simulink model "arducopter"  (R2021a)
settings: Solver=FixedStepAuto  StartTime=0.0  StopTime=simIn.param.timeEnd  FixedStep=simIn.param.dt  RelTol=1e-3
undefined symbols (not defined in the file or in its folder): DiscIntNeverNeededParam, sim, simIn
libraries: simulink x35, slident x4, vrlib x1
(part 8 of 9)

== matlab function arducopter/Lowpass2p/Lowpass Yaw/Lowpass2p ==
  data: u input; y output; sampleFreq input; cutoffFreq input; delElem1 data_store_memory; delElem2 data_store_memory
function y = lowpass2p(u, sampleFreq, cutoffFreq)
% Lowpass filter of order two
% Source: LowPassFilter2p.cpp
global delElem1
global delElem2

% Calculate parameters: LowPassFilter2p.cpp, compute_params()
fr = single(sampleFreq/cutoffFreq);
ohm = single(tan(pi/fr));
c = single(1+2*cos(pi/4)*ohm + ohm*ohm);

b0 = ohm*ohm/c;
b1 = 2*b0;
b2 = b0;
a1 = 2*(ohm*ohm-1)/c;
a2 = single((1-2*cos(pi/4)*ohm+ohm*ohm)/c);

% Calculation of filtered sample: LowPassFilter2p.cpp, apply()
delElem0 = u - delElem1 * a1 - delElem2 * a2;
y = delElem0 * b0 + delElem1 * b1 + delElem2 * b2;

delElem2 = delElem1;
delElem1 = delElem0;

== matlab function arducopter/Body Frame Rates -> DCM/MATLAB Function ==
  data: dcm input; quaternion output
function quaternion = from_rotation_matrix(dcm)
% Function to calculate quaternion from a given rotation matrix.
% Implemented based on QuaternionT<T>::from_rotation_matrx()

m00 = dcm(1,1);
m11 = dcm(2,2);
m22 = dcm(3,3);
m10 = dcm(2,1);
m01 = dcm(1,2);
m20 = dcm(3,1);
m02 = dcm(1,3);
m21 = dcm(3,2);
m12 = dcm(2,3);

tr = m00 + m11 + m22;

if tr > 0
    S = sqrt(tr+1) * 2;
    qw = 0.25 * S;
    qx = (m21 - m12) / S;
    qy = (m02 - m20) / S;
    qz = (m10 - m01) / S;
elseif ((m00 > m11) && (m00 > m22))
    S = sqrt(1.0 + m00 - m11 - m22) * 2.0;
    qw = (m21 - m12) / S;
    qx = 0.25 * S;
    qy = (m01 + m10) / S;
    qz = (m02 + m20) / S;
elseif (m11 > m22)
    S = sqrt(1.0 + m11 - m00 - m22) * 2.0;
    qw = (m02 - m20) / S;
    qx = (m01 + m10) / S;
    qy = 0.25 * S;
    qz = (m12 + m21) / S;
else
    S = sqrt(1.0 + m22 - m00 - m11) * 2.0;
    qw = (m10 - m01) / S;
    qx = (m02 + m20) / S;
    qy = (m12 + m21) / S;
    qz = 0.25 * S;
end

quaternion = [qw;qx;qy;qz];

== matlab function arducopter/Attitude Controller/MATLAB Function ==
  data: rollIn input; rollOut output; pitchIn input; angleMax input; angleLimit input; pitchOut output; rpyInputMax input
function [rollOut, pitchOut] = get_pilot_desired_lean_angles(rollIn, pitchIn, angleMax, angleLimit, rpyInputMax)
% Code based on Mode::get_pilot_desired_lean_angles()
% Transform pilot's roll and pitch input into desired lean angle in
% centi-degrees

% Calculate inputs to rc_input_to_roll_pitch() function
rollInUnit = rollIn / rpyInputMax;
pitchInUnit = pitchIn / rpyInputMax;
angleMax = angleMax / 100;
angleLimit = angleLimit / 100;

%% The following lines result from the call to rc_input_to_roll_pitch() (control.cpp)
angleMaxDeg = min(angleMax, 85);
rc2rad = angleMaxDeg * pi / 180;

% Convert roll and pitch stick positions to normalized horizontal thrust
thrust_x = -1 * tan(rc2rad * pitchInUnit);
thrust_y = tan(rc2rad * rollInUnit);

% Calculate the horizontal thrust limit based on the angle limit
angleLimit = min( max( 10, angleLimit), angleMaxDeg);
thrustLimit = tan(angleLimit * pi / 180);

% Apply horizontal thrust limit - Lines are taken from
% Vector2<T>::limit_length() and limit thrust vector norm
thrustVecLength = sqrt(thrust_x^2 + thrust_y^2);
if thrustVecLength > thrustLimit && thrustVecLength > 0
   thrust_x = thrust_x * (thrustLimit / thrustVecLength);
   thrust_y = thrust_y * (thrustLimit / thrustVecLength);
end

% Conversion from angular thrust to euler angles
pitchRad = (-1) * atan(thrust_x);
rollRad = atan(cos(pitchRad) * thrust_y);

% Output values in centi-degrees
pitchOut = pitchRad * (100 * 180) / pi;
rollOut = rollRad * (100 * 180) / pi;

== matlab function arducopter/Attitude Controller/MATLAB Function1 ==
  data: yawIn input; yawOut output; pilotYawExpo input; pilotYawRate input
function yawOut = get_pilot_desired_yaw_rate(yawIn, pilotYawExpo, pilotYawRate)
% Code taken from Mode::get_pilot_desired_yaw_rate()
% Transforms pilot's yaw input into a desired yaw rate

%% 1) Apply expo - Code based on input_expo in control.cpp
yawIn = min(max(yawIn, -1), 1);
if pilotYawExpo < 0.95
    yawIn = (1 - pilotYawExpo) * yawIn / (1 - pilotYawExpo * abs(yawIn));
end

%% 2) Convert pilot input to the desired yaw rate
yawOut = pilotYawRate * 100 * yawIn;

== matlab function arducopter/Attitude Controller/input_euler_angle_roll_pitch_euler_rate_yaw()/MATLAB Function ==
  data: q input; roll output; pitch output; yaw output
function [roll, pitch, yaw] = toEuler(q)
% Function takes a quaternion and translates it into Euler angles
% Based on QuaternionT<T>::to_euler() and incorporates 
% QuaternionT<T>::get_euler_roll(), QuaternionT<T>::get_euler_pitch() and
% QuaternionT<T>::get_euler_yaw()

roll = single(atan2(2 * (q(1)*q(2) + q(3)*q(4)), 1 - 2*(q(2)*q(2) + q(3)*q(3))));
% Check if argument of asin is greater than 1 oder smaller than -1
% Based on safe_asin() in AP_MATH.cpp
xPitch = 2 * (q(1)*q(3) - q(4)*q(2));
if xPitch >= 1
    pitch = single(pi/2);
elseif xPitch <= -1
    pitch = single(-pi/2);
else
    pitch = single(asin(xPitch));
end
yaw = single(atan2(2*(q(1)*q(4) + q(2)*q(3)), 1 - 2*(q(3)*q(3) + q(4)*q(4))));

== matlab function arducopter/Attitude Controller/input_euler_angle_roll_pitch_euler_rate_yaw()/Feedforward enabled/MATLAB Function ==
  data: eulerAngleTar input; eulerAccelMaxBF output; eulerAccelMaxEF input
function eulerAccelMaxBF = euler_accel_limit(eulerAngleTar, eulerAccelMaxEF)
% Translation of acceleration limits eulerAccelMax to the euler axis
% Code based on AC_AttitudeControl::euler_accel_limit()

sin_phi = max(min(abs(single(sin(eulerAngleTar(1)))), 1), 0.1); % Sinus of roll angle
cos_phi = max(min(abs(single(cos(eulerAngleTar(1)))), 1), 0.1);
sin_theta = max(min(abs(single(sin(eulerAngleTar(2)))), 1), 0.1); % Sinus of pitch angle

eulerAccelMaxBF = single(zeros(3,1));
if eulerAccelMaxEF(1) == 0 || eulerAccelMaxEF(2) == 0 || eulerAccelMaxEF(3) == 0 || ...
   eulerAccelMaxEF(1) < 0 || eulerAccelMaxEF(2) < 0 || eulerAccelMaxEF(3) < 0 
    eulerAccelMaxBF(1) = eulerAccelMaxEF(1);
    eulerAccelMaxBF(2) = eulerAccelMaxEF(2);
    eulerAccelMaxBF(3) = eulerAccelMaxEF(3);
else
    eulerAccelMaxBF(1) = eulerAccelMaxEF(1);
    eulerAccelMaxBF(2) = min(eulerAccelMaxEF(2) / cos_phi, eulerAccelMaxEF(3) / sin_phi);
    eulerAccelMaxBF(3) = min(min(eulerAccelMaxEF(1) / sin_theta, eulerAccelMaxEF(2) / sin_phi), eulerAccelMaxEF(3) / cos_phi);
end

== matlab function arducopter/Attitude Controller/input_euler_angle_roll_pitch_euler_rate_yaw()/Feedforward enabled/input shaping/input shaping roll angle/Square Root Controller ==
  data: err input; correction_rate output; p input; second_ord_lim input; dt input
function correction_rate = sqrt_controller(err, p, second_ord_lim, dt)
% The square root controller
% Code is taken from sqrt_controller(...) in AC_PosControl.cpp, line 296.

if (second_ord_lim < 0 || second_ord_lim == 0)
   correction_rate = err * p;
elseif (p == 0)
    % P term is zero, but second order limit is positive
    if (err > 0)
        correction_rate = sqrt(single(2.0) * second_ord_lim * err);
    elseif (err < 0)
        correction_rate = sqrt(single(2.0) * second_ord_lim * -err);
    else
        correction_rate = single(0.0);
    end
else
    % P term and second order limit are positive, hence have been defined
    linear_dist = second_ord_lim / (p * p);
    % Check if error exceeds linear range of controller gain
    if (err > linear_dist)
        correction_rate = sqrt(single(2.0) * second_ord_lim * ( err - (linear_dist / single(2.0)) ));
    elseif (err < -linear_dist)
        correction_rate = -sqrt(single(2.0) * second_ord_lim * ( -err - (linear_dist / single(2.0)) ));
    else
        % Return linearly amplified correction if error is in linear range
        correction_rate = err * p;
    end
end

% Prevent oscillations by over-shooting the error correction in the last
% time step
if (dt ~= 0)
    correction_rate = max( min(correction_rate, abs(err) / dt), -abs(err) / dt);
end

== matlab function arducopter/Attitude Controller/input_euler_angle_roll_pitch_euler_rate_yaw()/Feedforward enabled/input shaping/input shaping roll angle/MATLAB Function ==
  data: radIn input; radLim output
function radLim = wrapPi(radIn)
% Function to limit input angle in radian to [-pi pi].
% Code based on wrap_PI() and wrap_2PI() of AP_Math.cpp

% 1) Limit to [0 2pi]
radLim = mod(radIn, 2*pi);
if radLim < 0
    radLim = radLim + 2*pi;
end

% 2) Limit to [0 pi]
if radLim > pi
    radLim = radLim - 2*pi;
end

== matlab function arducopter/Attitude Controller/input_euler_angle_roll_pitch_euler_rate_yaw()/Feedforward enabled/input shaping/input shaping roll angle/MATLAB Function1 ==
  data: desiredAngVel input; targetAngVel input; eulerRateTar output; accelMax input; dt input; input_tc input
function eulerRateTar = input_shaping_ang_vel(desiredAngVel, targetAngVel, accelMax, dt, input_tc)
% Limits acceleration and deceleration of a velocity request
% Code based on AC_AttitudeControl::input_shaping_ang_vel()

if input_tc > 0
    % Calculate the acceleration to smoothly achieve rate. Jerk is not limited.
    errorRate = desiredAngVel - targetAngVel;
    desiredAngAccel = sqrt_controller(errorRate, 1.0/max(input_tc, single(0.01)), single(0), dt);
    desiredAngVel = targetAngVel + desiredAngAccel * dt;
end

% Acceleration is limited directly to smooth the beginning of the curve
if accelMax > 0
    deltaAngVel = accelMax * dt;
    eulerRateTar = min(max(desiredAngVel, targetAngVel - deltaAngVel), targetAngVel + deltaAngVel);
else
    eulerRateTar = desiredAngVel;
end

== matlab function arducopter/Attitude Controller/input_euler_angle_roll_pitch_euler_rate_yaw()/Feedforward enabled/input shaping/input shaping pitch angle/MATLAB Function ==
  data: radIn input; radLim output
function radLim = wrapPi(radIn)
% Function to limit input angle in radian to [-pi pi].
% Code based on wrap_PI() and wrap_2PI() of AP_Math.cpp

% 1) Limit to [0 2pi]
radLim = mod(radIn, 2*pi);
if radLim < 0
    radLim = radLim + 2*pi;
end

% 2) Limit to [0 pi]
if radLim > pi
    radLim = radLim - 2*pi;
end

== matlab function arducopter/Attitude Controller/input_euler_angle_roll_pitch_euler_rate_yaw()/reset yaw targets/MATLAB Function9 ==
  data: q1 input; qRes output; q2 input
function qRes = quatMult(q1, q2)
% Quaternion multiplication. Code based on QuaternionT<T>::operator*() in
% quaternion.cpp

qRes = single(zeros(4,1));
qRes(1) = q1(1)*q2(1) - q1(2)*q2(2) - q1(3)*q2(3) - q1(4)*q2(4);
qRes(2) = q1(1)*q2(2) + q1(2)*q2(1) + q1(3)*q2(4) - q1(4)*q2(3);
qRes(3) = q1(1)*q2(3) - q1(2)*q2(4) + q1(3)*q2(1) + q1(4)*q2(2);
qRes(4) = q1(1)*q2(4) + q1(2)*q2(3) - q1(3)*q2(2) + q1(4)*q2(1);

== matlab function arducopter/Attitude Controller/input_euler_angle_roll_pitch_euler_rate_yaw()/Feedforward enabled/input shaping/input shaping pitch angle/Square Root Controller ==
  data: err input; correction_rate output; p input; second_ord_lim input; dt input
function correction_rate = sqrt_controller(err, p, second_ord_lim, dt)
% The square root controller
% Code is taken from sqrt_controller(...) in AC_PosControl.cpp, line 296.

if (second_ord_lim < 0 || second_ord_lim == 0)
   correction_rate = err * p;
elseif (p == 0)
    % P term is zero, but second order limit is positive
    if (err > 0)
        correction_rate = sqrt(single(2.0) * second_ord_lim * err);
    elseif (err < 0)
        correction_rate = sqrt(single(2.0) * second_ord_lim * -err);
    else
        correction_rate = single(0.0);
    end
else
    % P term and second order limit are positive, hence have been defined
    linear_dist = second_ord_lim / (p * p);
    % Check if error exceeds linear range of controller gain
    if (err > linear_dist)
        correction_rate = sqrt(single(2.0) * second_ord_lim * ( err - (linear_dist / single(2.0)) ));
    elseif (err < -linear_dist)
        correction_rate = -sqrt(single(2.0) * second_ord_lim * ( -err - (linear_dist / single(2.0)) ));
    else
        % Return linearly amplified correction if error is in linear range
        correction_rate = err * p;
    end
end

% Prevent oscillations by over-shooting the error correction in the last
% time step
if (dt ~= 0)
    correction_rate = max( min(correction_rate, abs(err) / dt), -abs(err) / dt);
end

== matlab function arducopter/Rate Controller/PID Pitch Rate/I/Integrator ==
  data: error input; integrator_out output; integrator input single; limit_flg input; ki input; i_max input; dt input
function integrator_out = fcn(error, integrator, limit_flg, ki, i_max, dt)
% Code is based on AC_PID::update_i() in AC_PID.cpp.

% Check plausibility of input parameters
if (ki ~= 0 && dt > 0)
    % Only allow integration if limit is not set or the absolute sum of the
    % integrator would be reduced.
    if (~limit_flg || (integrator > 0 && error < 0) || (integrator < 0 && error > 0))
        integrator_out = integrator + error * ki * dt;
        integrator_out = max( min(integrator_out, i_max), -i_max);
    else % Otherwise, keep old integrator value
        integrator_out = integrator;
    end
else % Reset integrator if input parameters are not plausible
    integrator_out = single(0.0);
end

== matlab function arducopter/Attitude Controller/input_euler_angle_roll_pitch_euler_rate_yaw()/Feedforward enabled/MATLAB Function1 ==
  data: eulerAngle input; angVelTar output; eulerRate input
function angVelTar = euler_rate_to_ang_vel(eulerAngle, eulerRate)
% This function converts euler angle derivatives (321 system) to an angular
% velocity vector. eulerAngle is the vector of the euler angles in rad and
% eulerRate is the vector of euler rates in rad/s
% Code based on AC_AttitudeControl::euler_rate_to_ang_vel()

sin_theta = single(sin(eulerAngle(2)));
cos_theta = single(cos(eulerAngle(2)));
sin_phi = single(sin(eulerAngle(1)));
cos_phi = single(cos(eulerAngle(1)));

angVelTar = single(zeros(3,1));
angVelTar(1) = eulerRate(1) - sin_theta * eulerRate(3);
angVelTar(2) = cos_phi * eulerRate(2) + sin_phi * cos_theta * eulerRate(3);
angVelTar(3) = -sin_phi * eulerRate(2) + cos_theta * cos_phi * eulerRate(3);

== matlab function arducopter/Attitude Controller/input_euler_angle_roll_pitch_euler_rate_yaw()/reset yaw targets/MATLAB Function1 ==
  data: q input; roll output; pitch output; yaw output
function [roll, pitch, yaw] = toEuler(q)
% Function takes a quaternion and translates it into Euler angles
% Based on QuaternionT<T>::to_euler() and incorporates 
% QuaternionT<T>::get_euler_roll(), QuaternionT<T>::get_euler_pitch() and
% QuaternionT<T>::get_euler_yaw()

roll = single(atan2(2 * (q(1)*q(2) + q(3)*q(4)), 1 - 2*(q(2)*q(2) + q(3)*q(3))));
% Check if argument of asin is greater than 1 oder smaller than -1
% Based on safe_asin() in AP_MATH.cpp
xPitch = 2 * (q(1)*q(3) - q(4)*q(2));
if xPitch >= 1
    pitch = single(pi/2);
elseif xPitch <= -1
    pitch = single(-pi/2);
else
    pitch = single(asin(xPitch));
end
yaw = single(atan2(2*(q(1)*q(4) + q(2)*q(3)), 1 - 2*(q(3)*q(3) + q(4)*q(4))));

== matlab function arducopter/Attitude Controller/input_euler_angle_roll_pitch_euler_rate_yaw()/Feedforward enabled/MATLAB Function2 ==
  data: angVelTar input; angVelTarLimited output; angVelRollMax input; angVelPitchMax input; angVelYawMax input
function angVelTarLimited = ang_vel_limit(angVelTar, angVelRollMax, angVelPitchMax, angVelYawMax)
% Limits angular velocity (rad/s) in body frame
% Code based on AC_AttitudeControl::ang_vel_limit()

angVelTarLimited = angVelTar;
if angVelRollMax == 0 || angVelPitchMax == 0
    if angVelRollMax ~= 0
        angVelTarLimited(1) = max(min(angVelTar(1), angVelRollMax), -angVelRollMax);
    end
    if angVelPitchMax ~= 0
        angVelTarLimited(2) = max(min(angVelTar(2), angVelPitchMax), -angVelPitchMax);
    end
else
    thrustVecAngVel = [angVelTar(1) / angVelRollMax; angVelTar(2) / angVelPitchMax];
    thrustVecLen = single(sqrt(thrustVecAngVel(1)^2 + thrustVecAngVel(2)^2));
    if thrustVecLen > 1
        angVelTarLimited(1) = thrustVecAngVel(1) * angVelRollMax / thrustVecLen;
        angVelTarLimited(2) = thrustVecAngVel(2) * angVelPitchMax / thrustVecLen;
    end
end
if angVelYawMax ~= 0
    angVelTarLimited(3) = max(min(angVelTar(3), angVelYawMax), -angVelYawMax);
end

== matlab function arducopter/Attitude Controller/input_euler_angle_roll_pitch_euler_rate_yaw()/Feedforward enabled/MATLAB Function3 ==
  data: angVelBf input; eulerAngle input; eulerRate output
function eulerRate = ang_vel_to_euler_rate(angVelBf,eulerAngle)
% Function converts body-frame angular velocity into euler rate of desired
% attitude
% Based on AC_AttitudeControl::ang_vel_to_euler_rate()

sin_theta = single(sin(eulerAngle(2)));
cos_theta = single(cos(eulerAngle(2)));
sin_phi = single(sin(eulerAngle(1)));
cos_phi = single(cos(eulerAngle(1)));

eulerRate = single(zeros(3,1));
eulerRate(1) = angVelBf(1) + sin_phi * (sin_theta / cos_theta) * angVelBf(2) + cos_phi * (sin_theta / cos_theta) * angVelBf(3);
eulerRate(2) = cos_phi * angVelBf(2) - sin_phi * angVelBf(3);
eulerRate(3) = (sin_phi / cos_theta) * angVelBf(2) + (cos_phi / cos_theta) * angVelBf(3);

== matlab function arducopter/Attitude Controller/input_euler_angle_roll_pitch_euler_rate_yaw()/Feedforward disabled/MATLAB Function ==
  data: roll input; q output; pitch input; yaw input
function q = fromEuler(roll, pitch, yaw)
% Computes quaternion from euler angle vector
% Based on QuaternionT<T>::from_euler()

q = single(zeros(4,1));
cr2 = single(cos(roll*0.5));
cp2 = single(cos(pitch*0.5));
cy2 = single(cos(yaw*0.5));
sr2 = single(sin(roll*0.5));
sp2 = single(sin(pitch*0.5));
sy2 = single(sin(yaw*0.5));

q(1) = cr2*cp2*cy2 + sr2*sp2*sy2;
q(2) = sr2*cp2*cy2 - cr2*sp2*sy2;
q(3) = cr2*sp2*cy2 + sr2*cp2*sy2;
q(4) = cr2*cp2*sy2 - sr2*sp2*cy2;

== matlab function arducopter/Attitude Controller/input_euler_angle_roll_pitch_euler_rate_yaw()/thrust_heading_rotation_angles()/thrust_vector_rotation_angles()/MATLAB Function ==
  data: q input; vecRot output; vec input
function vecRot = rotateByQuat(q, vec)
% Function rotates vector vec by quaternion q. Equivalent to converting the
% input quaternion to a rotation matrix and then multiplying it by the
% vector. This uses the formula
%
%    v2 = v1 + 2 q1 * qv x v1 + 2 qv x qv x v1
%
% where "x" is the cross product (explicitly inlined for performance below), 
% "q1" is the scalar part and "qv" is the vector part of this quaternion
% Code based on Vector3<T> QuaternionT<T>::operator*()

vecRot = vec;

% Compute and cache "qv x v1"
uv = [q(3) * vec(3) - q(4) * vec(2); q(4) * vec(1) - q(2) * vec(3); q(2) * vec(2) - q(3) * vec(1)];

uv(1) = uv(1) + uv(1);
uv(2) = uv(2) + uv(2);
uv(3) = uv(3) + uv(3);
vecRot(1) = vecRot(1) + q(1) * uv(1) + q(3) * uv(3) - q(4) * uv(2);
vecRot(2) = vecRot(2) + q(1) * uv(2) + q(4) * uv(1) - q(2) * uv(3);
vecRot(3) = vecRot(3) + q(1) * uv(3) + q(2) * uv(2) - q(3) * uv(1);

== matlab function arducopter/Attitude Controller/input_euler_angle_roll_pitch_euler_rate_yaw()/thrust_heading_rotation_angles()/thrust_vector_rotation_angles()/MATLAB Function1 ==
  data: q input; vecRot output; vec input
function vecRot = rotateByQuat(q, vec)
% Function rotates vector vec by quaternion q. Equivalent to converting the
% input quaternion to a rotation matrix and then multiplying it by the
% vector. This uses the formula
%
%    v2 = v1 + 2 q1 * qv x v1 + 2 qv x qv x v1
%
% where "x" is the cross product (explicitly inlined for performance below), 
% "q1" is the scalar part and "qv" is the vector part of this quaternion
% Code based on Vector3<T> QuaternionT<T>::operator*()

vecRot = vec;

% Compute and cache "qv x v1"
uv = [q(3) * vec(3) - q(4) * vec(2); q(4) * vec(1) - q(2) * vec(3); q(2) * vec(2) - q(3) * vec(1)];

uv(1) = uv(1) + uv(1);
uv(2) = uv(2) + uv(2);
uv(3) = uv(3) + uv(3);
vecRot(1) = vecRot(1) + q(1) * uv(1) + q(3) * uv(3) - q(4) * uv(2);
vecRot(2) = vecRot(2) + q(1) * uv(2) + q(4) * uv(1) - q(2) * uv(3);
vecRot(3) = vecRot(3) + q(1) * uv(3) + q(2) * uv(2) - q(3) * uv(1);

== matlab function arducopter/Attitude Controller/input_euler_angle_roll_pitch_euler_rate_yaw()/thrust_heading_rotation_angles()/thrust_vector_rotation_angles()/MATLAB Function2 ==
  data: thrustErrAngle input; rotVec input; rotVecNorm output
function rotVecNorm = normalizeVec(thrustErrAngle, rotVec)
% Function to normalize the thrust rotation vector. Divides the vector by
% its length or uses up-vector if thrust error angle is zero
rotVecNorm = single(zeros(3,1));
vecLen = single(sqrt(rotVec(1)^2 + rotVec(2)^2 + rotVec(3)^2));

if thrustErrAngle == 0 || vecLen == 0
    rotVecNorm = single([0;0;-1]);
else
    rotVecNorm(1) = rotVec(1) / vecLen;
    rotVecNorm(2) = rotVec(2) / vecLen;
    rotVecNorm(3) = rotVec(3) / vecLen;
end

== matlab function arducopter/Attitude Controller/input_euler_angle_roll_pitch_euler_rate_yaw()/thrust_heading_rotation_angles()/thrust_vector_rotation_angles()/MATLAB Function3 ==
  data: q input; qInv output
function qInv = invertQuat(q)
% Function inverts the rotation of a quaternion.
% Code based on QuaternionT<T>::inverse(void)
% qInv = [q(1);-q(2);-q(3);-q(4)];
qInv = single(zeros(4,1));
qInv(1) = q(1);
qInv(2) = -q(2);
qInv(3) = -q(3);
qInv(4) = -q(4);

== matlab function arducopter/Attitude Controller/input_euler_angle_roll_pitch_euler_rate_yaw()/thrust_heading_rotation_angles()/thrust_vector_rotation_angles()/MATLAB Function4 ==
  data: q input; vecRot output; vec input
function vecRot = rotateByQuat(q, vec)
% Function rotates vector vec by quaternion q. Equivalent to converting the
% input quaternion to a rotation matrix and then multiplying it by the
% vector. This uses the formula
%
%    v2 = v1 + 2 q1 * qv x v1 + 2 qv x qv x v1
%
% where "x" is the cross product (explicitly inlined for performance below), 
% "q1" is the scalar part and "qv" is the vector part of this quaternion
% Code based on Vector3<T> QuaternionT<T>::operator*()

vecRot = vec;

% Compute and cache "qv x v1"
uv = [q(3) * vec(3) - q(4) * vec(2); q(4) * vec(1) - q(2) * vec(3); q(2) * vec(2) - q(3) * vec(1)];

uv(1) = uv(1) + uv(1);
uv(2) = uv(2) + uv(2);
uv(3) = uv(3) + uv(3);
vecRot(1) = vecRot(1) + q(1) * uv(1) + q(3) * uv(3) - q(4) * uv(2);
vecRot(2) = vecRot(2) + q(1) * uv(2) + q(4) * uv(1) - q(2) * uv(3);
vecRot(3) = vecRot(3) + q(1) * uv(3) + q(2) * uv(2) - q(3) * uv(1);

== matlab function arducopter/Attitude Controller/input_euler_angle_roll_pitch_euler_rate_yaw()/thrust_heading_rotation_angles()/thrust_vector_rotation_angles()/MATLAB Function5 ==
  data: axis input; angle input; q output
function q = fromAxisAngle(axis, angle)
% Create a quaternion from its axis-angle representation. The axis-vector
% must be of length 1 and the angle in radians.
% Based on QuaternionT<T>::from_axis_angle()

q = single(zeros(4,1));

if angle == 0
    q(1) = 1;
    q(2) = 0;
    q(3) = 0;
    q(4) = 0;
else
    st2 = sin(0.5*angle);
    q(1) = cos(0.5*angle);
    q(2) = axis(1) * st2;
    q(3) = axis(2) * st2;
    q(4) = axis(3) * st2;
end

== matlab function arducopter/Attitude Controller/input_euler_angle_roll_pitch_euler_rate_yaw()/thrust_heading_rotation_angles()/thrust_vector_rotation_angles()/MATLAB Function6 ==
  data: q input; vec output single
function vec = toAxisAngle(q)
% Converts the quaternion to a rotation vector. The direction represents
% the axis of rotation and the length represents the angle of rotation
% Code based on QuaternionT<T>::to_axis_angle()
l = sqrt(q(2)^2 + q(3)^2 + q(4)^2);

vec = [q(2);q(3);q(4)];

if l ~= 0
    vec = vec ./ l;
    mult = 2 * atan2(l, q(1));
    % The following lines are taken from wrap_pi() in AP_Math.cpp
    mult = mod(mult, 2*pi);
    if mult < 0
        mult = mult + 2*pi;
    end
    if mult > pi
        mult = mult - 2*pi;
    end

    vec = vec .* mult;
end

== matlab function arducopter/Attitude Controller/input_euler_angle_roll_pitch_euler_rate_yaw()/thrust_heading_rotation_angles()/thrust_vector_rotation_angles()/MATLAB Function7 ==
  data: q input; qInv output
function qInv = invertQuat(q)
% Function inverts the rotation of a quaternion.
% Code based on QuaternionT<T>::inverse(void)
% qInv = [q(1);-q(2);-q(3);-q(4)];
qInv = single(zeros(4,1));
qInv(1) = q(1);
qInv(2) = -q(2);
qInv(3) = -q(3);
qInv(4) = -q(4);

== matlab function arducopter/Attitude Controller/input_euler_angle_roll_pitch_euler_rate_yaw()/thrust_heading_rotation_angles()/thrust_vector_rotation_angles()/MATLAB Function8 ==
  data: q input; qInv output
function qInv = invertQuat(q)
% Function inverts the rotation of a quaternion.
% Code based on QuaternionT<T>::inverse(void)
qInv = [q(1);-q(2);-q(3);-q(4)];

== matlab function arducopter/Attitude Controller/input_euler_angle_roll_pitch_euler_rate_yaw()/thrust_heading_rotation_angles()/thrust_vector_rotation_angles()/MATLAB Function9 ==
  data: q1 input; qRes output; q2 input
function qRes = quatMult(q1, q2)
% Quaternion multiplication. Code based on QuaternionT<T>::operator*() in
% quaternion.cpp

qRes = single(zeros(4,1));
qRes(1) = q1(1)*q2(1) - q1(2)*q2(2) - q1(3)*q2(3) - q1(4)*q2(4);
qRes(2) = q1(1)*q2(2) + q1(2)*q2(1) + q1(3)*q2(4) - q1(4)*q2(3);
qRes(3) = q1(1)*q2(3) - q1(2)*q2(4) + q1(3)*q2(1) + q1(4)*q2(2);
qRes(4) = q1(1)*q2(4) + q1(2)*q2(3) - q1(3)*q2(2) + q1(4)*q2(1);

== matlab function arducopter/Throttle/Throttle Calculations/Boost and Premixing/Throttle_In Handling ==
  data: thrTar input; angBst input; thrHover input; thrOut output; angBstEna input; thrAvgMax output single; thrRpyMix input
function [thrOut, thrAvgMax] = fcn(thrTar, angBst, thrHover, angBstEna, thrRpyMix)
% The following lines represent the set_throttle_out() function in
% AC_AttitudeControl_Multi.cpp, that takes the desired throttle from the
% pilot and calculate the boosted and average max throttle.
if(angBstEna)
    % Reference: AC_AttitudeControl_Multi::get_throttle_boosted(throttle_in)
    thrOut = thrTar + angBst;
else
    thrOut = thrTar;
end

%% Determine throttle_avg_max
thr_des_max = max(thrOut, thrTar);

% The following lines are taken from get_throttle_avg_max()
% Limit throttle_max to [0,1]
thr_des_max = min( max( thr_des_max, single(0)), single(1));

% Calculate maximum throttle between input throttle and needed throttle
% considering mix between roll/pitch and hovering
thrAvgMax = max(thr_des_max, thr_des_max * max( single(0), (single(1)-thrRpyMix) ) + thrHover * thrRpyMix);

== matlab function arducopter/Attitude Controller/input_euler_angle_roll_pitch_euler_rate_yaw()/thrust_heading_rotation_angles()/thrust_vector_rotation_angles()/MATLAB Function10 ==
  data: q input; vec output single
function vec = toAxisAngle(q)
% Converts the quaternion to a rotation vector. The direction represents
% the axis of rotation and the length represents the angle of rotation
% Code based on QuaternionT<T>::to_axis_angle()
l = sqrt(q(2)^2 + q(3)^2 + q(4)^2);

vec = [q(2);q(3);q(4)];

if l ~= 0
    vec = vec ./ l;
    mult = 2 * atan2(l, q(1));
    % The following lines are taken from wrap_pi() in AP_Math.cpp
    mult = mod(mult, 2*pi);
    if mult < 0
        mult = mult + 2*pi;
    end
    if mult > pi
        mult = mult - 2*pi;
    end

    vec = vec .* mult;
end

== matlab function arducopter/Attitude Controller/input_euler_angle_roll_pitch_euler_rate_yaw()/thrust_heading_rotation_angles()/thrust_vector_rotation_angles()/MATLAB Function11 ==
  data: q1 input; qRes output; q2 input
function qRes = quatMult(q1, q2)
% Quaternion multiplication. Code based on QuaternionT<T>::operator*() in
% quaternion.cpp

qRes = single(zeros(4,1));
qRes(1) = q1(1)*q2(1) - q1(2)*q2(2) - q1(3)*q2(3) - q1(4)*q2(4);
qRes(2) = q1(1)*q2(2) + q1(2)*q2(1) + q1(3)*q2(4) - q1(4)*q2(3);
qRes(3) = q1(1)*q2(3) - q1(2)*q2(4) + q1(3)*q2(1) + q1(4)*q2(2);
qRes(4) = q1(1)*q2(4) + q1(2)*q2(3) - q1(3)*q2(2) + q1(4)*q2(1);

== matlab function arducopter/Attitude Controller/input_euler_angle_roll_pitch_euler_rate_yaw()/thrust_heading_rotation_angles()/thrust_vector_rotation_angles()/MATLAB Function12 ==
  data: q1 input; qRes output; q2 input
function qRes = quatMult(q1, q2)
% Quaternion multiplication. Code based on QuaternionT<T>::operator*() in
% quaternion.cpp

qRes = single(zeros(4,1));
qRes(1) = q1(1)*q2(1) - q1(2)*q2(2) - q1(3)*q2(3) - q1(4)*q2(4);
qRes(2) = q1(1)*q2(2) + q1(2)*q2(1) + q1(3)*q2(4) - q1(4)*q2(3);
qRes(3) = q1(1)*q2(3) - q1(2)*q2(4) + q1(3)*q2(1) + q1(4)*q2(2);
qRes(4) = q1(1)*q2(4) + q1(2)*q2(3) - q1(3)*q2(2) + q1(4)*q2(1);

== matlab function arducopter/Attitude Controller/input_euler_angle_roll_pitch_euler_rate_yaw()/thrust_heading_rotation_angles()/thrust_vector_rotation_angles()/MATLAB Function13 ==
  data: q input; qInv output
function qInv = invertQuat(q)
% Function inverts the rotation of a quaternion.
% Code based on QuaternionT<T>::inverse(void)
qInv = [q(1);-q(2);-q(3);-q(4)];

== matlab function arducopter/Attitude Controller/input_euler_angle_roll_pitch_euler_rate_yaw()/thrust_heading_rotation_angles()/thrust_vector_rotation_angles()/MATLAB Function14 ==
  data: q input; qInv output
function qInv = invertQuat(q)
% Function inverts the rotation of a quaternion.
% Code based on QuaternionT<T>::inverse(void)
qInv = [q(1);-q(2);-q(3);-q(4)];

== matlab function arducopter/Attitude Controller/input_euler_angle_roll_pitch_euler_rate_yaw()/thrust_heading_rotation_angles()/thrust_vector_rotation_angles()/MATLAB Function15 ==
  data: q1 input; qRes output; q2 input
function qRes = quatMult(q1, q2)
% Quaternion multiplication. Code based on QuaternionT<T>::operator*() in
% quaternion.cpp

qRes = single(zeros(4,1));
qRes(1) = q1(1)*q2(1) - q1(2)*q2(2) - q1(3)*q2(3) - q1(4)*q2(4);
qRes(2) = q1(1)*q2(2) + q1(2)*q2(1) + q1(3)*q2(4) - q1(4)*q2(3);
qRes(3) = q1(1)*q2(3) - q1(2)*q2(4) + q1(3)*q2(1) + q1(4)*q2(2);
qRes(4) = q1(1)*q2(4) + q1(2)*q2(3) - q1(3)*q2(2) + q1(4)*q2(1);

== matlab function arducopter/Attitude Controller/input_euler_angle_roll_pitch_euler_rate_yaw()/thrust_heading_rotation_angles()/thrust_vector_rotation_angles()/MATLAB Function16 ==
  data: q input; vec output
function vec = toAxisAngle(q)
% Converts the quaternion to a rotation vector. The direction represents
% the axis of rotation and the length represents the angle of rotation
% Code based on QuaternionT<T>::to_axis_angle()
l = sqrt(q(2)^2 + q(3)^2 + q(4)^2);

vec = [q(2);q(3);q(4)];

if l ~= 0
    vec = vec ./ l;
    mult = 2 * atan2(l, q(1));
    % The following lines are taken from wrap_pi() in AP_Math.cpp
    mult = mod(mult, 2*pi);
    if mult < 0
        mult = mult + 2*pi;
    end
    if mult > pi
        mult = mult - 2*pi;
    end

    vec = vec .* mult;
end

== matlab function arducopter/Attitude Controller/input_euler_angle_roll_pitch_euler_rate_yaw()/thrust_heading_rotation_angles()/Yaw error limitation/Yaw limiting and recalculation of attitudeTarget/MATLAB Function ==
  data: radIn input; radLim output
function radLim = wrapPi(radIn)
% Function to limit input angle in radian to [-pi pi].
% Code based on wrap_PI() and wrap_2PI() of AP_Math.cpp

% 1) Limit to [0 2pi]
radLim = mod(radIn, 2*pi);
if radLim < 0
    radLim = radLim + 2*pi;
end

% 2) Limit to [0 pi]
if radLim > pi
    radLim = radLim - 2*pi;
end

== matlab function arducopter/Attitude Controller/input_euler_angle_roll_pitch_euler_rate_yaw()/thrust_heading_rotation_angles()/Yaw error limitation/Yaw limiting and recalculation of attitudeTarget/MATLAB Function5 ==
  data: vec input; q output
function q = fromAxisAngle(vec)
% Create a quaternion from its axis-angle representation. Just the rotation
% vector is given as input.
% Based on QuaternionT<T>::from_axis_angle(Vector3<T>)

q = single(zeros(4,1));
angle = sqrt(vec(1)^2 + vec(2)^2 + vec(3)^2);

if angle == 0
    q(1) = 1;
    q(2) = 0;
    q(3) = 0;
    q(4) = 0;
else
    axis = vec ./ angle;
    % The following lines are based on QuaternionT<T>::from_axis_angle(const Vector3<T> &axis, T theta)
    if angle == 0
        q(1) = 1;
        q(2) = 0;
        q(3) = 0;
        q(4) = 0;
    else
        st2 = sin(0.5*angle);
        q(1) = cos(0.5*angle);
        q(2) = axis(1) * st2;
        q(3) = axis(2) * st2;
        q(4) = axis(3) * st2;
    end
end

== matlab function arducopter/Attitude Controller/input_euler_angle_roll_pitch_euler_rate_yaw()/thrust_heading_rotation_angles()/Yaw error limitation/Yaw limiting and recalculation of attitudeTarget/MATLAB Function9 ==
  data: q1 input; qRes output; q2 input
function qRes = quatMult(q1, q2)
% Quaternion multiplication. Code based on QuaternionT<T>::operator*() in
% quaternion.cpp

qRes = single(zeros(4,1));
qRes(1) = q1(1)*q2(1) - q1(2)*q2(2) - q1(3)*q2(3) - q1(4)*q2(4);
qRes(2) = q1(1)*q2(2) + q1(2)*q2(1) + q1(3)*q2(4) - q1(4)*q2(3);
qRes(3) = q1(1)*q2(3) - q1(2)*q2(4) + q1(3)*q2(1) + q1(4)*q2(2);
qRes(4) = q1(1)*q2(4) + q1(2)*q2(3) - q1(3)*q2(2) + q1(4)*q2(1);

== matlab function arducopter/Attitude Controller/input_euler_angle_roll_pitch_euler_rate_yaw()/thrust_heading_rotation_angles()/Yaw error limitation/Yaw limiting and recalculation of attitudeTarget/MATLAB Function1 ==
  data: q1 input; qRes output; q2 input
function qRes = quatMult(q1, q2)
% Quaternion multiplication. Code based on QuaternionT<T>::operator*() in
% quaternion.cpp

qRes = single(zeros(4,1));
qRes(1) = q1(1)*q2(1) - q1(2)*q2(2) - q1(3)*q2(3) - q1(4)*q2(4);
qRes(2) = q1(1)*q2(2) + q1(2)*q2(1) + q1(3)*q2(4) - q1(4)*q2(3);
qRes(3) = q1(1)*q2(3) - q1(2)*q2(4) + q1(3)*q2(1) + q1(4)*q2(2);
qRes(4) = q1(1)*q2(4) + q1(2)*q2(3) - q1(3)*q2(2) + q1(4)*q2(1);

== matlab function arducopter/Attitude Controller/input_euler_angle_roll_pitch_euler_rate_yaw()/update_ang_vel_target_from_att_error()/Calc angular velocity target roll/Square Root Controller ==
  data: err input; correction_rate output; p input; second_ord_lim input; dt input
function correction_rate = sqrt_controller(err, p, second_ord_lim, dt)
% The square root controller
% Code is taken from sqrt_controller(...) in AC_PosControl.cpp, line 296.

if (second_ord_lim < 0 || second_ord_lim == 0)
   correction_rate = err * p;
elseif (p == 0)
    % P term is zero, but second order limit is positive
    if (err > 0)
        correction_rate = sqrt(single(2.0) * second_ord_lim * err);
    elseif (err < 0)
        correction_rate = sqrt(single(2.0) * second_ord_lim * -err);
    else
        correction_rate = single(0.0);
    end
else
    % P term and second order limit are positive, hence have been defined
    linear_dist = second_ord_lim / (p * p);
    % Check if error exceeds linear range of controller gain
    if (err > linear_dist)
        correction_rate = sqrt(single(2.0) * second_ord_lim * ( err - (linear_dist / single(2.0)) ));
    elseif (err < -linear_dist)
        correction_rate = -sqrt(single(2.0) * second_ord_lim * ( -err - (linear_dist / single(2.0)) ));
    else
        % Return linearly amplified correction if error is in linear range
        correction_rate = err * p;
    end
end

% Prevent oscillations by over-shooting the error correction in the last
% time step
if (dt ~= 0)
    correction_rate = max( min(correction_rate, abs(err) / dt), -abs(err) / dt);
end

== matlab function arducopter/Attitude Controller/input_euler_angle_roll_pitch_euler_rate_yaw()/update_ang_vel_target_from_att_error()/Calc angular velocity target pitch/Square Root Controller ==
  data: err input; correction_rate output; p input; second_ord_lim input; dt input
function correction_rate = sqrt_controller(err, p, second_ord_lim, dt)
% The square root controller
% Code is taken from sqrt_controller(...) in AC_PosControl.cpp, line 296.

if (second_ord_lim < 0 || second_ord_lim == 0)
   correction_rate = err * p;
elseif (p == 0)
    % P term is zero, but second order limit is positive
    if (err > 0)
        correction_rate = sqrt(single(2.0) * second_ord_lim * err);
    elseif (err < 0)
        correction_rate = sqrt(single(2.0) * second_ord_lim * -err);
    else
        correction_rate = single(0.0);
    end
else
    % P term and second order limit are positive, hence have been defined
    linear_dist = second_ord_lim / (p * p);
    % Check if error exceeds linear range of controller gain
    if (err > linear_dist)
        correction_rate = sqrt(single(2.0) * second_ord_lim * ( err - (linear_dist / single(2.0)) ));
    elseif (err < -linear_dist)
        correction_rate = -sqrt(single(2.0) * second_ord_lim * ( -err - (linear_dist / single(2.0)) ));
    else
        % Return linearly amplified correction if error is in linear range
        correction_rate = err * p;
    end
end

% Prevent oscillations by over-shooting the error correction in the last
% time step
if (dt ~= 0)
    correction_rate = max( min(correction_rate, abs(err) / dt), -abs(err) / dt);
end

== matlab function arducopter/Attitude Controller/input_euler_angle_roll_pitch_euler_rate_yaw()/update_ang_vel_target_from_att_error()/Calc angular velocity target yaw/Square Root Controller ==
  data: err input; correction_rate output; p input; second_ord_lim input; dt input
function correction_rate = sqrt_controller(err, p, second_ord_lim, dt)
% The square root controller
% Code is taken from sqrt_controller(...) in AC_PosControl.cpp, line 296.

if (second_ord_lim < 0 || second_ord_lim == 0)
   correction_rate = err * p;
elseif (p == 0)
    % P term is zero, but second order limit is positive
    if (err > 0)
        correction_rate = sqrt(single(2.0) * second_ord_lim * err);
    elseif (err < 0)
        correction_rate = sqrt(single(2.0) * second_ord_lim * -err);
    else
        correction_rate = single(0.0);
    end
else
    % P term and second order limit are positive, hence have been defined
    linear_dist = second_ord_lim / (p * p);
    % Check if error exceeds linear range of controller gain
    if (err > linear_dist)
        correction_rate = sqrt(single(2.0) * second_ord_lim * ( err - (linear_dist / single(2.0)) ));
    elseif (err < -linear_dist)
        correction_rate = -sqrt(single(2.0) * second_ord_lim * ( -err - (linear_dist / single(2.0)) ));
    else
        % Return linearly amplified correction if error is in linear range
        correction_rate = err * p;
    end
end

% Prevent oscillations by over-shooting the error correction in the last
% time step
if (dt ~= 0)
    correction_rate = max( min(correction_rate, abs(err) / dt), -abs(err) / dt);
end

== matlab function arducopter/Attitude Controller/input_euler_angle_roll_pitch_euler_rate_yaw()/MATLAB Function2 ==
  data: angVel input; angVelLimited output; angVelRollMax input; angVelPitchMax input; angVelYawMax input
function angVelLimited = ang_vel_limit(angVel, angVelRollMax, angVelPitchMax, angVelYawMax)
% Limits angular velocity (rad/s) in body frame
% Code based on AC_AttitudeControl::ang_vel_limit()

angVelLimited = angVel;
if angVelRollMax == 0 || angVelPitchMax == 0
    if angVelRollMax ~= 0
        angVelLimited(1) = max(min(angVel(1), angVelRollMax), -angVelRollMax);
    end
    if angVelPitchMax ~= 0
        angVelLimited(2) = max(min(angVel(2), angVelPitchMax), -angVelPitchMax);
    end
else
    thrustVecAngVel = [angVel(1) / angVelRollMax; angVel(2) / angVelPitchMax];
    thrustVecLen = single(sqrt(thrustVecAngVel(1)^2 + thrustVecAngVel(2)^2));
    if thrustVecLen > 1
        angVelLimited(1) = thrustVecAngVel(1) * angVelRollMax / thrustVecLen;
        angVelLimited(2) = thrustVecAngVel(2) * angVelPitchMax / thrustVecLen;
    end
end
if angVelYawMax ~= 0
    angVelLimited(3) = max(min(angVel(3), angVelYawMax), -angVelYawMax);
end

== matlab function arducopter/Throttle/Throttle Calculations/Throttle-Attitude-Mixing/Update Throttle Mix ==
  data: thrMixDes input; thrMix output; thrMixMin input; thrMixMax input; thrOut input; thrIn input; thrHover input; dt input; thrMixAct data_store_memory
function thrMix = updateThrMix(thrMixDes, thrMixMin, thrMixMax, thrOut, thrIn, thrHover, dt)
% The function represents the update_throttle_rpy_mix() function in
% AC_AttitudeControl_Multi.cpp
% The function slowly moves rpy_mix to rpy_mix_des which represents the
% desired mix between hover and thrust throttle.
global thrMixAct

if thrMixAct < thrMixDes
    thrMix = thrMixAct + min(2 * dt, thrMixDes - thrMixAct);
elseif thrMixAct > thrMixDes
    thrMix = thrMixAct - min(0.5 * dt, thrMixAct - thrMixDes);
    
    % If the mix is still higher than that being used, reset immediately
    thrOut = max(thrOut, thrIn);
    % since thrOut >= thrIn at this point, we dont't need to
    % check thrIn < thrHover
    if thrOut < thrHover
        mixUsed = (thrOut - thrIn) / (thrHover - thrIn);
    else
        mixUsed = thrOut / thrHover;
    end
    
    thrMix = min(thrMix, max(mixUsed, thrMixDes));
else   % Added else statement due to compiler error for uninitialized output
    thrMix = thrMixAct;
end

thrMix = max( min( thrMix, thrMixMax), thrMixMin );

== matlab function arducopter/Attitude Controller/input_euler_angle_roll_pitch_euler_rate_yaw()/MATLAB Function7 ==
  data: q input; qInv output
function qInv = invertQuat(q)
% Function inverts the rotation of a quaternion.
% Code based on QuaternionT<T>::inverse(void)
% qInv = [q(1);-q(2);-q(3);-q(4)];
qInv = single(zeros(4,1));
qInv(1) = q(1);
qInv(2) = -q(2);
qInv(3) = -q(3);
qInv(4) = -q(4);

== matlab function arducopter/Attitude Controller/input_euler_angle_roll_pitch_euler_rate_yaw()/MATLAB Function11 ==
  data: q1 input; qRes output; q2 input
function qRes = quatMult(q1, q2)
% Quaternion multiplication. Code based on QuaternionT<T>::operator*() in
% quaternion.cpp

qRes = single(zeros(4,1));
qRes(1) = q1(1)*q2(1) - q1(2)*q2(2) - q1(3)*q2(3) - q1(4)*q2(4);
qRes(2) = q1(1)*q2(2) + q1(2)*q2(1) + q1(3)*q2(4) - q1(4)*q2(3);
qRes(3) = q1(1)*q2(3) - q1(2)*q2(4) + q1(3)*q2(1) + q1(4)*q2(2);
qRes(4) = q1(1)*q2(4) + q1(2)*q2(3) - q1(3)*q2(2) + q1(4)*q2(1);

== matlab function arducopter/Attitude Controller/input_euler_angle_roll_pitch_euler_rate_yaw()/MATLAB Function4 ==
  data: q input; vecRot output; vec input
function vecRot = rotateByQuat(q, vec)
% Function rotates vector vec by quaternion q. Equivalent to converting the
% input quaternion to a rotation matrix and then multiplying it by the
% vector. This uses the formula
%
%    v2 = v1 + 2 q1 * qv x v1 + 2 qv x qv x v1
%
% where "x" is the cross product (explicitly inlined for performance below), 
% "q1" is the scalar part and "qv" is the vector part of this quaternion
% Code based on Vector3<T> QuaternionT<T>::operator*()

vecRot = vec;

% Compute and cache "qv x v1"
uv = [q(3) * vec(3) - q(4) * vec(2); q(4) * vec(1) - q(2) * vec(3); q(2) * vec(2) - q(3) * vec(1)];

uv(1) = uv(1) + uv(1);
uv(2) = uv(2) + uv(2);
uv(3) = uv(3) + uv(3);
vecRot(1) = vecRot(1) + q(1) * uv(1) + q(3) * uv(3) - q(4) * uv(2);
vecRot(2) = vecRot(2) + q(1) * uv(2) + q(4) * uv(1) - q(2) * uv(3);
vecRot(3) = vecRot(3) + q(1) * uv(3) + q(2) * uv(2) - q(3) * uv(1);

== matlab function arducopter/Attitude Controller/input_euler_angle_roll_pitch_euler_rate_yaw()/Add feedforward to angVelBody/MATLAB Function ==
  data: angVelBodyFeedforward input; angVelBodyNew output; angVelBodyIn input; thrustErrorAngle input; yawRateAct input; maxThrustErrorAngle4YawCorr input; feedforwardScaler output
function [angVelBodyNew, feedforwardScaler] = addFeedforwardToTargetAngVel(angVelBodyFeedforward, angVelBodyIn, thrustErrorAngle, yawRateAct, maxThrustErrorAngle4YawCorr)
% Function smoothly adds feedforward angular velocity and yaw input to
% target angular velocity.
% Code based on AC_AttitudeControl::attitude_controller_run_quat()

angVelBodyNew = angVelBodyIn;

feedforwardScaler = single(1);
if thrustErrorAngle > 2 * maxThrustErrorAngle4YawCorr
    % thrustErrorAngle too large. Set target yaw rate to actual rate. Do not
    % add feedforward.
    angVelBodyNew(3) = yawRateAct;
elseif thrustErrorAngle > maxThrustErrorAngle4YawCorr
    % thrustErrorAngle still large. Add feedforward values smoothly.
    feedforwardScaler = 1 - (thrustErrorAngle - maxThrustErrorAngle4YawCorr) / maxThrustErrorAngle4YawCorr;
    angVelBodyNew(1) = angVelBodyNew(1) + angVelBodyFeedforward(1) * feedforwardScaler;
    angVelBodyNew(2) = angVelBodyNew(2) + angVelBodyFeedforward(2) * feedforwardScaler;
    angVelBodyNew(3) = angVelBodyNew(3) + angVelBodyFeedforward(3);
    angVelBodyNew(3) = yawRateAct * (1 - feedforwardScaler) + angVelBodyNew(3) * feedforwardScaler;
else
    % thrustErrorAngle small enough to add feedforward values to target
    % angular rates of controller without smoothing.
    angVelBodyNew = angVelBodyNew + angVelBodyFeedforward;
end

== matlab function arducopter/Attitude Controller/input_euler_angle_roll_pitch_euler_rate_yaw()/Update attitudeTarget/MATLAB Function ==
  data: q input; qNorm output
function qNorm = normalizeQuat(q)
% Function to normalze a quaternion. Code based on
% QuaternionT<T>::normalize()

quatLen = single(sqrt(q(1)^2 + q(2)^2 + q(3)^2 + q(4)^2));
if quatLen ~= 0
    qNorm = q ./ quatLen;
else
    qNorm = q;
end

== matlab function arducopter/Attitude Controller/input_euler_angle_roll_pitch_euler_rate_yaw()/Update attitudeTarget/Rotate target attitude/MATLAB Function5 ==
  data: vec input; q output
function q = fromAxisAngle(vec)
% Create a quaternion from its axis-angle representation. Just the rotation
% vector is given as input.
% Based on QuaternionT<T>::from_axis_angle(Vector3<T>)

q = zeros(4,1);
angle = single(sqrt(vec(1)^2 + vec(2)^2 + vec(3)^2));

if angle == 0
    q(1) = single(1);
    q(2) = single(0);
    q(3) = single(0);
    q(4) = single(0);
else
    axis = vec ./ angle;
    % The following lines are based on QuaternionT<T>::from_axis_angle(const Vector3<T> &axis, T theta)
    if angle == 0
        q(1) = single(1);
        q(2) = single(0);
        q(3) = single(0);
        q(4) = single(0);
    else
        st2 = single(sin(0.5*angle));
        q(1) = single(cos(0.5*angle));
        q(2) = axis(1) * st2;
        q(3) = axis(2) * st2;
        q(4) = axis(3) * st2;
    end
end

== matlab function arducopter/Attitude Controller/input_euler_angle_roll_pitch_euler_rate_yaw()/Update attitudeTarget/Rotate target attitude/MATLAB Function1 ==
  data: q1 input; qRes output; q2 input
function qRes = quatMult(q1, q2)
% Quaternion multiplication. Code based on QuaternionT<T>::operator*() in
% quaternion.cpp

qRes = single(zeros(4,1));
qRes(1) = q1(1)*q2(1) - q1(2)*q2(2) - q1(3)*q2(3) - q1(4)*q2(4);
qRes(2) = q1(1)*q2(2) + q1(2)*q2(1) + q1(3)*q2(4) - q1(4)*q2(3);
qRes(3) = q1(1)*q2(3) - q1(2)*q2(4) + q1(3)*q2(1) + q1(4)*q2(2);
qRes(4) = q1(1)*q2(4) + q1(2)*q2(3) - q1(3)*q2(2) + q1(4)*q2(1);

== matlab function arducopter/Body Frame Rates -> DCM/MATLAB Function1 ==
  data: rotMat input; roll output; pitch output; yaw output
function [roll, pitch, yaw] = to_euler(rotMat)
% Calculate euler angles from a rotation matrix
% Based on Matrix3<T>::to_euler()
cx = single(1);
pitch = single(0);
roll = single(0);
yaw = single(0);

if rotMat(3,1) >= 1
    cx = 2*single(pi);
end
if rotMat(3,1) <= -1
    cx = -2*single(pi);
else
    cx = rotMat(3,1);
end
pitch = -asin(cx);
roll = atan2(rotMat(3,2), rotMat(3,3));
yaw = atan2(rotMat(2,1), rotMat(1,1));

== matlab function arducopter/Body Frame Rates -> DCM/MATLAB Function2 ==
  data: roll input; rotMat output; pitch input; yaw input
function rotMat = fromEuler(roll, pitch, yaw)
% Computes rotation matrix from euler angle vector
% Based on QuaternionT<T>::from_euler()

rotMat = single(zeros(3,3));
cp = single(cos(pitch));
sp = single(sin(pitch));
sr = single(sin(roll));
cr = single(cos(roll));
sy = single(sin(yaw));
cy = single(cos(yaw));

rotMat(1,1) = cp * cy;
rotMat(1,2) = (sr * sp * cy) - (cr * sy);
rotMat(1,3) = (cr * sp * cy) + (sr * sy);
rotMat(2,1) = cp * sy;
rotMat(2,2) = (sr * sp * sy) + (cr * cy);
rotMat(2,3) = (cr * sp * sy) - (sr * cy);
rotMat(3,1) =  -sp;
rotMat(3,2) = sr * cp;
rotMat(3,3) = cr * cp;

== matlab function arducopter/Body Frame Rates -> DCM/MATLAB Function3 ==
  data: dcm input; quaternion output
function quaternion = from_rotation_matrix(dcm)
% Function to calculate quaternion from a given rotation matrix.
% Implemented based on QuaternionT<T>::from_rotation_matrx()

m00 = dcm(1,1);
m11 = dcm(2,2);
m22 = dcm(3,3);
m10 = dcm(2,1);
m01 = dcm(1,2);
m20 = dcm(3,1);
m02 = dcm(1,3);
m21 = dcm(3,2);
m12 = dcm(2,3);

tr = m00 + m11 + m22;

if tr > 0
    S = sqrt(tr+1) * 2;
    qw = 0.25 * S;
    qx = (m21 - m12) / S;
    qy = (m02 - m20) / S;
    qz = (m10 - m01) / S;
elseif ((m00 > m11) && (m00 > m22))
    S = sqrt(1.0 + m00 - m11 - m22) * 2.0;
    qw = (m21 - m12) / S;
    qx = 0.25 * S;
    qy = (m01 + m10) / S;
    qz = (m02 + m20) / S;
elseif (m11 > m22)
    S = sqrt(1.0 + m11 - m00 - m22) * 2.0;
    qw = (m02 - m20) / S;
    qx = (m01 + m10) / S;
    qy = 0.25 * S;
    qz = (m12 + m21) / S;
else
    S = sqrt(1.0 + m22 - m00 - m11) * 2.0;
    qw = (m10 - m01) / S;
    qx = (m02 + m20) / S;
    qy = (m12 + m21) / S;
    qz = 0.25 * S;
end

quaternion = [qw;qx;qy;qz];
